simulink model "SpeedGoatLoop_v3"  (R2020b)
settings: Solver=FixedStepAuto  StartTime=0.0  StopTime=60*60*1.5  RelTol=1e-3
libraries: fl_lib x42, nesl_utility x19, SimscapeFluids_lib x4, speedgoatlib_IO132 x2, slpidlib x2
(part 2 of 2)

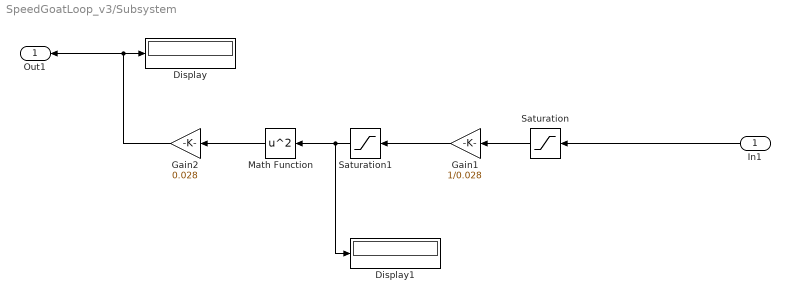
== system SpeedGoatLoop_v3/Subsystem ==
  In1 : Inport
  Display : Display
  Display1 : Display
  Gain1 : Gain  Gain=1/0.028
  Gain2 : Gain  Gain=0.028
  Math Function : Math  Operator=square  SaturateOnIntegerOverflow=on
  Saturation : Saturate  UpperLimit=20  LowerLimit=0
  Saturation1 : Saturate  UpperLimit=500  LowerLimit=0
  Out1 : Outport
  wires:
  In1/1 -> Saturation/1
  Saturation/1 -> Gain1/1
  Saturation1/1 -> Display1/1, Math Function/1
  Gain1/1 -> Saturation1/1
  Math Function/1 -> Gain2/1
  Gain2/1 -> Out1/1, Display/1

== matlab function SpeedGoatLoop_v3/MATLAB Function ==
  data: T input; dTdt output; valveCmd input; t input; Ts input; reset input; maxSlope output; ssThresh output; ssFlag output; ssTime output
function [dTdt, maxSlope, ssThresh, ssFlag, ssTime] = steadyStateMonitor(T, valveCmd, t, Ts, reset)
% valveCmd: 0 = closed, 1 = open
% reset: optional external reset

persistent Tprev maxSlopeLatch threshLatch ssTimer locked initialized firstRun

if isempty(initialized) || reset
    Tprev = T;
    maxSlopeLatch = 0;
    threshLatch = 0;
    ssTimer = 0;
    locked = false;
    initialized = true;
    
    firstRun = true;
end

% Discrete derivative
if firstRun
dTdt = 0;
firstRun = false;
else
    dTdt = (T- Tprev)/Ts;
end

Tprev = T;
%Ignore unrealistic startup spikes
if abs(dTdt) > 2
    dTdt = 0;
end

% Record max heating rate
%Ignore first 5 seconds to avoid initialization transient

if ~locked
    if t > 5 && t < 300
       if abs(dTdt) > maxSlopeLatch
           maxSlopeLatch = abs(dTdt);
       end
    elseif t >= 300
        if maxSlopeLatch > 0
        threshLatch = 0.01 * maxSlopeLatch;
        end
            locked = true;
    end
end

%Outputs
maxSlope = maxSlopeLatch;
ssThresh  = threshLatch;


% Duration under steady-state condition
if locked && abs(dTdt) <= ssThresh
    ssFlag = true;
    ssTimer = ssTimer + Ts;
else
    ssTimer = 0;   % change to "ssTimer = ssTimer + Ts;" if you want total time instead of consecutive time
    ssFlag = false;
end

ssTime = ssTimer;
end
